simulink model "nonlinear_pid"  (R2023b)
settings: Solver=VariableStepAuto  StartTime=0.0  StopTime=10.0  RelTol=1e-3
libraries: simulink_extras x1
settings Model: Creator=USER  LastModifiedBy=USER

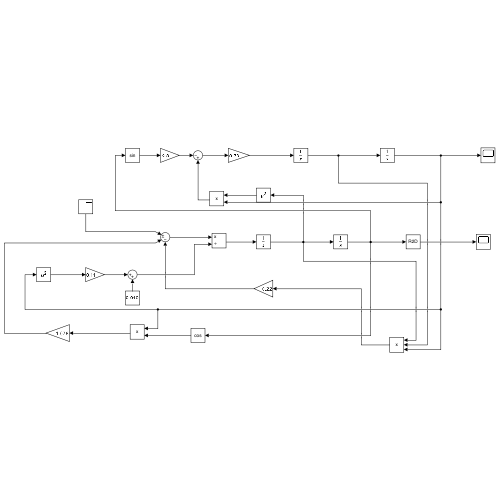
[thumbnail: Simulink's stored preview of the top-level diagram]
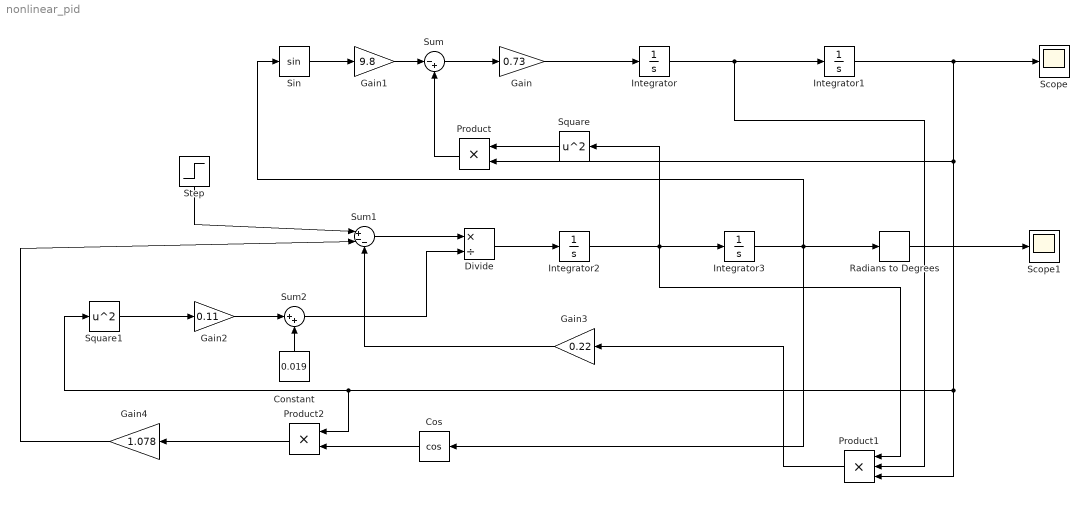
== system nonlinear_pid ==
  Constant : Constant  Value=0.019
  Cos : Trigonometry  Operator=cos
  Divide : Product  Inputs=*/
  Gain : Gain  Gain=0.73
  Gain1 : Gain  Gain=9.8
  Gain2 : Gain  Gain=0.11
  Gain3 : Gain  Gain=0.22
  Gain4 : Gain  Gain=1.078
  Integrator{,1..3} (4 alike) : Integrator
  Product : Product
  Product1 : Product  Inputs=3
  Product2 : Product
  Radians to Degrees : simulink_extras/Transformations/Radians to Degrees
  Scope : Scope
  Scope1 : Scope
  Sin : Trigonometry
  Square : Math  Operator=square
  Square1 : Math  Operator=square
  Step : Step  After=10*pi/180  SampleTime=0
  Sum : Sum  Inputs=|-+
  Sum1 : Sum  Inputs=|+--
  Sum2 : Sum  Inputs=|++
  wires:
  Gain2/1 -> Sum2/1
  Cos/1 -> Product2/2
  Gain3/1 -> Sum1/3
  Gain4/1 -> Sum1/2
  Sum/1 -> Gain/1
  Sin/1 -> Gain1/1
  Gain1/1 -> Sum/1
  Integrator3/1 -> Cos/1, Radians to Degrees/1, Sin/1
  Integrator1/1 -> Scope/1, Product/2, Product1/3, Square1/1, Product2/1
  Product1/1 -> Gain3/1
  Gain/1 -> Integrator/1
  Integrator/1 -> Integrator1/1, Product1/2
  Sum1/1 -> Divide/1
  Integrator2/1 -> Square/1, Integrator3/1, Product1/1
  Divide/1 -> Integrator2/1
  Product/1 -> Sum/2
  Sum2/1 -> Divide/2
  Constant/1 -> Sum2/2
  Radians to Degrees/1 -> Scope1/1
  Product2/1 -> Gain4/1
  Square/1 -> Product/1
  Square1/1 -> Gain2/1
  Step/1 -> Sum1/1
